simulink model "autogyro"  (R2025a)
settings: Solver=VariableStepAuto  StartTime=0.0  StopTime=100.0  RelTol=1e-3
values from neighbouring files (symbols this model uses):
  A = 0.005    [params.m]
  Cd = 0.47    [params.m]
  g = 9.81    [params.m]
  m = 1.3    [params.m]
  rho = 1.112    [params.m]
libraries: slpidlib x1
settings Model: Creator=Ana  LastModifiedBy=Ana

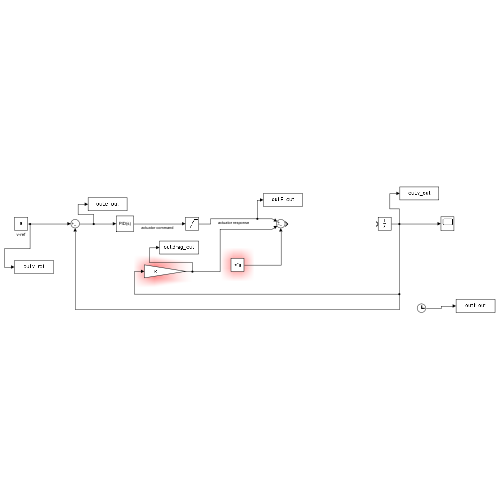
[thumbnail: Simulink's stored preview of the top-level diagram]
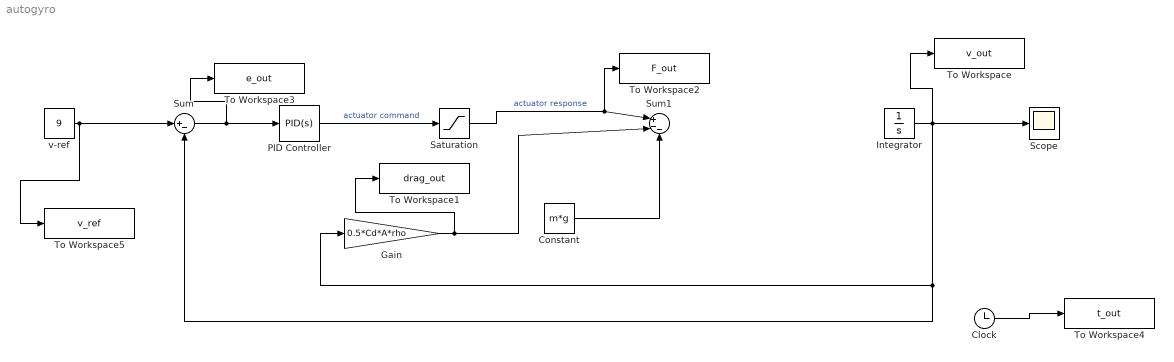
== system autogyro ==
  Clock : Clock
  Constant : Constant  Value=m*g
  Gain : Gain  Gain=0.5*Cd*A*rho
  Integrator : Integrator  InitialCondition=14
  PID Controller : slpidlib/PID Controller  Controller=PID  Form=Parallel  TimeDomain=Continuous-time  UseExternalTs=off  SampleTime=-1  IntegratorMethod=Forward Euler  FilterMethod=Forward Euler  ControllerParametersSource=internal  P=0.15550183173144  I=0.00347487197189414  UseKiTs=off  D=-0.505687454932131  UseExternalDerivativeSource=off  N=0.307505812562247  UseFilter=on  TunerSelectOption=Transfer Function Based (PID Tuner App)  InitialConditionSource=internal  InitialConditionForIntegrator=0  InitialConditionForFilter=0  DifferentiatorICPrevScaledInput=0  ExternalReset=none  TrackingMode=off  Kt=1  LimitOutput=off  SatLimitsSource=internal  UpperSaturationLimit=inf  LowerSaturationLimit=-inf  LinearizeAsGain=on  AntiWindupMode=none  Kb=1  LimitIntegrator=off  UpperIntegratorSaturationLimit=inf  LowerIntegratorSaturationLimit=-inf  POutMin=[]  POutMax=[]  IOutMin=[]  IOutMax=[]  DOutMin=[]  DOutMax=[]  NOutMin=[]  NOutMax=[]  SumOutMin=[]  SumOutMax=[]  SaturationOutMin=[]  SaturationOutMax=[]  PParamMin=[]  PParamMax=[]  IParamMin=[]  IParamMax=[]  DParamMin=[]  DParamMax=[]  NParamMin=[]  NParamMax=[]  KbParamMin=[]  KbParamMax=[]  KtParamMin=[]  KtParamMax=[]  KbOutMin=[]  KbOutMax=[]  KtOutMin=[]  KtOutMax=[]  IntegratorOutMin=[]  IntegratorOutMax=[]  FilterOutMin=[]  FilterOutMax=[]  SumI1OutMin=[]  SumI1OutMax=[]  SumI2OutMin=[]  SumI2OutMax=[]  SumI3OutMin=[]  SumI3OutMax=[]  SumI4OutMin=[]  SumI4OutMax=[]  SumDOutMin=[]  SumDOutMax=[]  DifferentiatorOutMin=[]  DifferentiatorOutMax=[]  FilterDiffOutCoefMin=[]  FilterDiffOutCoefMax=[]  ReciprocalOutMin=[]  ReciprocalOutMax=[]  SumDenOutMin=[]  SumDenOutMax=[]  SumNumOutMin=[]  SumNumOutMax=[]  DivideOutMin=[]  DivideOutMax=[]  UdiffTsProdOutMin=[]  UdiffTsProdOutMax=[]  NTsProdOutMin=[]  NTsProdOutMax=[]  UintegralTsProdOutMin=[]  UintegralTsProdOutMax=[]  UngainTsProdOutMin=[]  UngainTsProdOutMax=[]  ClampingZeroOutDataTypeStr=Inherit: Inherit via back propagation  ClampingZeroOutMin=[]  ClampingZeroOutMax=[]  FilterDenConstantOutDataTypeStr=Inherit: Inherit via back propagation  FilterDenConstantOutMin=[]  FilterDenConstantOutMax=[]  PCopyOutDataTypeStr=Inherit: Inherit via back propagation  PCopyOutMin=[]  PCopyOutMax=[]  NCopyOutDataTypeStr=Inherit: Inherit via back propagation  NCopyOutMin=[]  NCopyOutMax=[]  IntegratorContinuousStateAttributes=''  IntegratorStateMustResolveToSignalObject=off  IntegratorRTWStateStorageClass=Auto  FilterContinuousStateAttributes=''  FilterStateMustResolveToSignalObject=off  FilterRTWStateStorageClass=Auto  ParallelPVariant=InternalParameters  IdealPVariant=Disabled  IVariant=InternalParameters  DVariant=InternalParameters  IntegratorVariant=Continuous  SatVariant=Disabled  AWVariant=Passthrough  PCopyVariant=Disabled  TRVariant=Disabled  FdbkBlocksVariant=Forward  IdealPFdbkVariant=Disabled  SatFdbkVariant=Disabled  DerivativeFilterVariant=ContFilter  NVariant=InternalParameters  NCopyVariant=Disabled  FilterICVariant=InternalICsFilter  IntegratorICVariant=InternalICs  ExternalResetVariant=Disabled  TRSumVariant=Passthrough  SumFdbkVariant=Disabled  SumVariant=Sum_PID  TsampFilterVariant=InternalTs  TsampNgainVariant=Passthrough  TsampIntegralVariant=Disabled_SignalSpec  ExternalSaturationOutDataTypeStr=Inherit: Same as second input  DerivativeSourceVariant=ErrorSignal  PreIntVariant=InternalPreInt
  Saturation : Saturate  UpperLimit=30  LowerLimit=0
  Scope : Scope
      settings: ActiveDisplayYMinimum=1.8522967003407098  ActiveDisplayYMaximum=14.986211725799397
  Sum : Sum  Inputs=|+-
  Sum1 : Sum  Inputs=|+--
  To Workspace : ToWorkspace  VariableName=v_out  SampleTime=-1
  To Workspace1 : ToWorkspace  VariableName=drag_out  SampleTime=-1
  To Workspace2 : ToWorkspace  VariableName=F_out  SampleTime=-1
  To Workspace3 : ToWorkspace  VariableName=e_out  SampleTime=-1
  To Workspace4 : ToWorkspace  VariableName=t_out  SampleTime=-1
  To Workspace5 : ToWorkspace  VariableName=v_ref  SampleTime=-1
  v-ref : Constant  Value=9  VectorParams1D=off
  wires:
  v-ref/1 -> To Workspace5/1, Sum/1
  Sum/1 -> To Workspace3/1, PID Controller/1
  PID Controller/1 -> Saturation/1  "actuator command"
  Saturation/1 -> To Workspace2/1, Sum1/1  "actuator response"
  Constant/1 -> Sum1/3
  Gain/1 -> To Workspace1/1, Sum1/2
  Integrator/1 -> To Workspace/1, Scope/1, Sum/2, Gain/1
  Clock/1 -> To Workspace4/1
